simulink model "Mdl_FAST_IPC"  (R2023a)
settings: Solver=FixedStepAuto  StartTime=0.0  StopTime=10.0  FixedStep=DT  RelTol=1e-3
values from neighbouring files (symbols this model uses):
  wecs = 3.0    [DD_Mdl1.sldd]    (also in wecsmatfile.m = struct)
undefined symbols (not defined in the file or in its folder): OutList, strmatch
settings Model: DataDictionary=DD_Mdl1.sldd  Creator=ditt_aj  LastModifiedBy=jdi
settings SolverCC: AlgebraicLoopSolver=TrustRegion
settings DebuggingCC: UnconnectedInputMsg=warning  UnconnectedOutputMsg=warning  UnconnectedLineMsg=warning
settings ModelReferenceCC: EnableRefExpFcnMdlSchedulingChecks=on
settings SFSimCC: CustomCodeUndefinedFunction=UseInterfaceOnly
settings RTWCC: DLArmComputeVersion=19.05

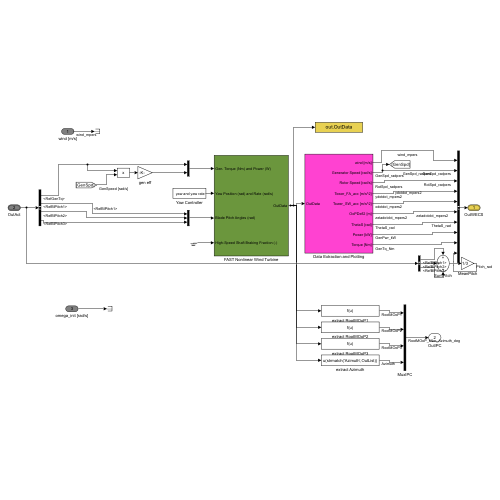
[thumbnail: Simulink's stored preview of the top-level diagram]
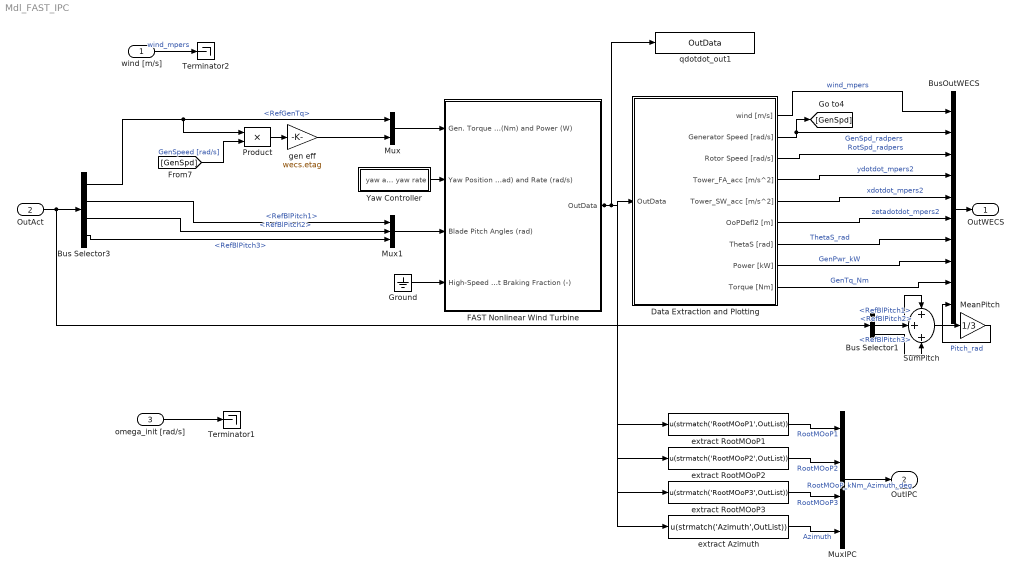
== system Mdl_FAST_IPC ==
  wind [m/s] : Inport
  OutAct : Inport  Port=2  OutDataTypeStr=Bus: slBus2
  omega_init [rad/s] : Inport  Port=3
  Bus Selector1 : BusSelector  OutputSignals=RefBlPitch1,RefBlPitch2,RefBlPitch3
  Bus Selector3 : BusSelector  OutputSignals=RefGenTq,RefBlPitch1,RefBlPitch2,RefBlPitch3
  BusOutWECS : BusCreator  Inputs=10  OutDataTypeStr=Bus: slBus1
  Data Extraction and Plotting : Subsystem
  FAST Nonlinear Wind Turbine : Subsystem  mask(FAST Nonlinear Wind Turbine){}
      mask help: This block contains the FAST S-Function.
      mask init:
      | clear FAST_SFunc
  Ground : Ground
  MeanPitch : Gain  Gain=1/3
  Mux : Mux  Inputs=2
  Mux1 : Mux  Inputs=3
  MuxIPC : Mux
  Product : Product  RndMeth=Zero
  SumPitch : Sum  Inputs=+++
  Terminator1 : Terminator
  Terminator2 : Terminator
  Yaw Controller : Subsystem
  extract Azimuth : Fcn  Expr=u(strmatch('Azimuth',OutList))
  extract RootMOoP1 : Fcn  Expr=u(strmatch('RootMOoP1',OutList))
  extract RootMOoP2 : Fcn  Expr=u(strmatch('RootMOoP2',OutList))
  extract RootMOoP3 : Fcn  Expr=u(strmatch('RootMOoP3',OutList))
  gen eff : Gain  Gain=wecs.etag
  qdotdot_out1 : ToWorkspace  VariableName=OutData  SampleTime=-1
  OutWECS : Outport  OutDataTypeStr=Bus: slBus1
  OutIPC : Outport  Port=2
  wires:
  Yaw Controller/1(yaw and yaw rate) -> FAST Nonlinear Wind Turbine/2(Yaw Position (rad) and Rate (rad/s))
  Ground/1 -> FAST Nonlinear Wind Turbine/4(High-Speed Shaft Braking Fraction (-))
  FAST Nonlinear Wind Turbine/1(OutData) -> qdotdot_out1/1, Data Extraction and Plotting/1(OutData), extract RootMOoP1/1, extract RootMOoP2/1, extract RootMOoP3/1, extract Azimuth/1
  Mux/1 -> FAST Nonlinear Wind Turbine/1(Gen. Torque (Nm) and Power (W))
  Mux1/1 -> FAST Nonlinear Wind Turbine/3(Blade Pitch Angles (rad))
  Product/1 -> gen eff/1
  [GenSpd] -> Product/2  "GenSpeed [rad/s]"
  gen eff/1 -> Mux/2
  omega_init [rad/s]/1 -> Terminator1/1
  Data Extraction and Plotting/6(OoPDefl2 [m]) -> BusOutWECS/6  "zetadotdot_mpers2"
  Bus Selector3/2 -> Mux1/1  "<RefBlPitch1>"
  Data Extraction and Plotting/3(Rotor Speed [rad/s]) -> BusOutWECS/3  "RotSpd_radpers"
  Data Extraction and Plotting/4(Tower_FA_acc [m/s^2]) -> BusOutWECS/4  "ydotdot_mpers2"
  Data Extraction and Plotting/7(ThetaS [rad]) -> BusOutWECS/7  "ThetaS_rad"
  Data Extraction and Plotting/2(Generator Speed [rad/s]) -> [GenSpd], BusOutWECS/2  "GenSpd_radpers"
  BusOutWECS/1 -> OutWECS/1
  Data Extraction and Plotting/5(Tower_SW_acc [m/s^2]) -> BusOutWECS/5  "xdotdot_mpers2"
  Data Extraction and Plotting/8(Power [kW]) -> BusOutWECS/8  "GenPwr_kW"
  Data Extraction and Plotting/9(Torque [Nm]) -> BusOutWECS/9  "GenTq_Nm"
  OutAct/1 -> Bus Selector1/1, Bus Selector3/1
  Bus Selector3/1 -> Product/1, Mux/1  "<RefGenTq>"
  Bus Selector3/3 -> Mux1/2  "<RefBlPitch2>"
  Bus Selector3/4 -> Mux1/3  "<RefBlPitch3>"
  wind [m/s]/1 -> Terminator2/1  "wind_mpers"
  Data Extraction and Plotting/1(wind [m/s]) -> BusOutWECS/1  "wind_mpers"
  extract RootMOoP1/1 -> MuxIPC/1  "RootMOoP1"
  extract RootMOoP2/1 -> MuxIPC/2  "RootMOoP2"
  extract RootMOoP3/1 -> MuxIPC/3  "RootMOoP3"
  extract Azimuth/1 -> MuxIPC/4  "Azimuth"
  MuxIPC/1 -> OutIPC/1  "RootMOoP_kNm_Azimuth_deg"
  Bus Selector1/1 -> SumPitch/1  "<RefBlPitch1>"
  Bus Selector1/2 -> SumPitch/2  "<RefBlPitch2>"
  Bus Selector1/3 -> SumPitch/3  "<RefBlPitch3>"
  SumPitch/1 -> MeanPitch/1
  MeanPitch/1 -> BusOutWECS/10  "Pitch_rad"

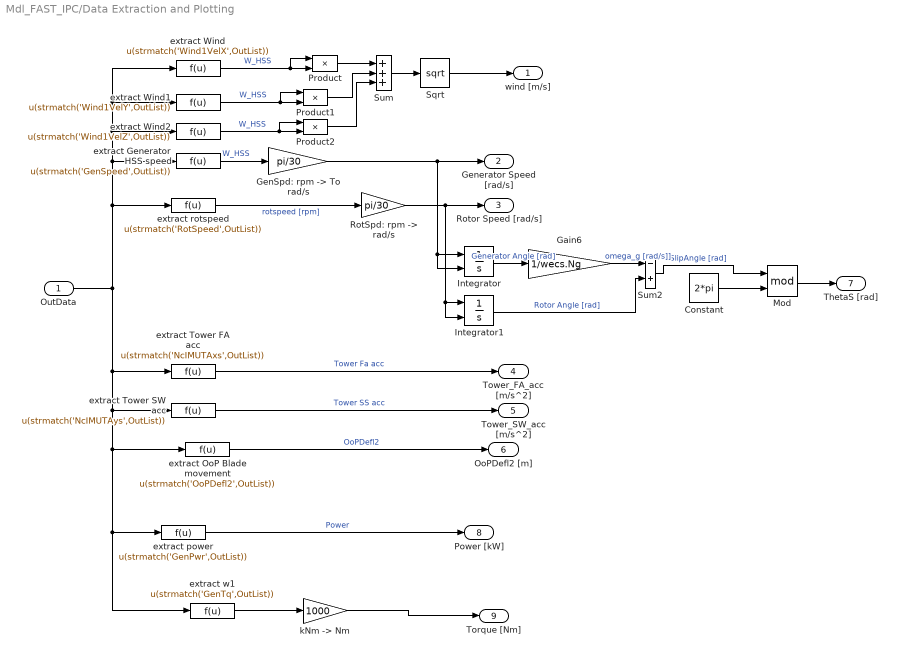
== system Mdl_FAST_IPC/Data Extraction and Plotting ==
  OutData : Inport
  Constant : Constant  Value=2*pi
  Gain6 : Gain  Gain=1/wecs.Ng
  "GenSpd: rpm -> To rad/s" : Gain  Gain=pi/30
  Integrator : Integrator  InitialConditionSource=external
  Integrator1 : Integrator  InitialConditionSource=external
  Mod : Math  Operator=mod
  Product : Product
  Product1 : Product
  Product2 : Product
  "RotSpd: rpm -> rad/s" : Gain  Gain=pi/30
  Sqrt : Sqrt
  Sum : Sum  Inputs=+++
  Sum2 : Sum  Inputs=-+
  extract Generator HSS speed : Fcn  Expr=u(strmatch('GenSpeed',OutList))
  extract OoP Blade movement : Fcn  Expr=u(strmatch('OoPDefl2',OutList))
  extract Tower FA acc : Fcn  Expr=u(strmatch('NcIMUTAxs',OutList))
  extract Tower SW acc : Fcn  Expr=u(strmatch('NcIMUTAys',OutList))
  extract Wind : Fcn  Expr=u(strmatch('Wind1VelX',OutList))
  extract Wind1 : Fcn  Expr=u(strmatch('Wind1VelY',OutList))
  extract Wind2 : Fcn  Expr=u(strmatch('Wind1VelZ',OutList))
  extract power : Fcn  Expr=u(strmatch('GenPwr',OutList))
  extract rotspeed : Fcn  Expr=u(strmatch('RotSpeed',OutList))
  extract w1 : Fcn  Expr=u(strmatch('GenTq',OutList))
  "kNm -> Nm" : Gain  Gain=1000
  wind [m/s] : Outport  VectorParamsAs1DForOutWhenUnconnected=off
  Generator Speed [rad/s] : Outport  Port=2  VectorParamsAs1DForOutWhenUnconnected=off
  Rotor Speed [rad/s] : Outport  Port=3  VectorParamsAs1DForOutWhenUnconnected=off
  Tower_FA_acc [m/s^2] : Outport  Port=4  VectorParamsAs1DForOutWhenUnconnected=off
  Tower_SW_acc [m/s^2] : Outport  Port=5  VectorParamsAs1DForOutWhenUnconnected=off
  OoPDefl2 [m] : Outport  Port=6  VectorParamsAs1DForOutWhenUnconnected=off
  ThetaS [rad] : Outport  Port=7  VectorParamsAs1DForOutWhenUnconnected=off
  Power [kW] : Outport  Port=8  VectorParamsAs1DForOutWhenUnconnected=off
  Torque [Nm] : Outport  Port=9  VectorParamsAs1DForOutWhenUnconnected=off
  wires:
  extract rotspeed/1 -> "RotSpd: rpm -> rad/s"/1  "rotspeed [rpm]"
  extract power/1 -> Power [kW]/1  "Power"
  extract Tower FA acc/1 -> Tower_FA_acc [m/s^2]/1  "Tower Fa acc"
  extract Tower SW acc/1 -> Tower_SW_acc [m/s^2]/1  "Tower SS acc"
  extract w1/1 -> "kNm -> Nm"/1
  "kNm -> Nm"/1 -> Torque [Nm]/1
  "RotSpd: rpm -> rad/s"/1 -> Integrator1/2, Integrator1/1, Rotor Speed [rad/s]/1
  "GenSpd: rpm -> To rad/s"/1 -> Integrator/2, Integrator/1, Generator Speed [rad/s]/1
  extract Generator HSS speed/1 -> "GenSpd: rpm -> To rad/s"/1  "W_HSS"
  extract OoP Blade movement/1 -> OoPDefl2 [m]/1  "OoPDefl2"
  OutData/1 -> extract power/1, extract w1/1, extract OoP Blade movement/1, extract Tower SW acc/1, extract Tower FA acc/1, extract Wind2/1, extract Wind1/1, extract Wind/1, extract Generator HSS speed/1, extract rotspeed/1
  Integrator/1 -> Gain6/1  "Generator Angle [rad]"
  Integrator1/1 -> Sum2/2  "Rotor Angle [rad]"
  Sum2/1 -> Mod/1  "SlipAngle [rad]"
  Constant/1 -> Mod/2
  Mod/1 -> ThetaS [rad]/1
  Gain6/1 -> Sum2/1  "omega_g [rad/s]]"
  extract Wind/1 -> Product/1, Product/2  "W_HSS"
  extract Wind1/1 -> Product1/1, Product1/2  "W_HSS"
  extract Wind2/1 -> Product2/1, Product2/2  "W_HSS"
  Product/1 -> Sum/1
  Product1/1 -> Sum/2
  Product2/1 -> Sum/3
  Sum/1 -> Sqrt/1
  Sqrt/1 -> wind [m/s]/1

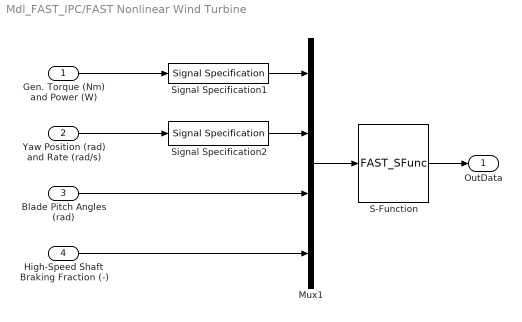
== system Mdl_FAST_IPC/FAST Nonlinear Wind Turbine ==
  Gen. Torque (Nm) and Power (W) : Inport
  Yaw Position (rad) and Rate (rad/s) : Inport  Port=2
  Blade Pitch Angles (rad) : Inport  Port=3
  High-Speed Shaft Braking Fraction (-) : Inport  Port=4
  Mux1 : Mux
  S-Function : S-Function  FunctionName=FAST_SFunc  Parameters=FAST_InputFileName, TMax, 0  SFunctionDeploymentMode=off  EnableBusSupport=off
  Signal Specification1 : SignalSpecification  OutDataTypeStr=double  Dimensions=2
  Signal Specification2 : SignalSpecification  OutDataTypeStr=double  Dimensions=2
  OutData : Outport  VectorParamsAs1DForOutWhenUnconnected=off
  wires:
  Gen. Torque (Nm) and Power (W)/1 -> Signal Specification1/1
  S-Function/1 -> OutData/1
  Mux1/1 -> S-Function/1
  Blade Pitch Angles (rad)/1 -> Mux1/3
  Yaw Position (rad) and Rate (rad/s)/1 -> Signal Specification2/1
  Signal Specification1/1 -> Mux1/1
  Signal Specification2/1 -> Mux1/2
  High-Speed Shaft Braking Fraction (-)/1 -> Mux1/4

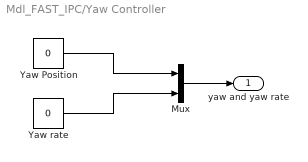
== system Mdl_FAST_IPC/Yaw Controller ==
  Mux : Mux  Inputs=2
  Yaw Position : Constant  Value=0
  Yaw rate : Constant  Value=0
  yaw and yaw rate : Outport  VectorParamsAs1DForOutWhenUnconnected=off
  wires:
  Mux/1 -> yaw and yaw rate/1
  Yaw Position/1 -> Mux/1
  Yaw rate/1 -> Mux/2
